simulink model "Sensores_Reales_2"  (R2026b)
settings: Solver=VariableStepAuto
values from neighbouring files (symbols this model uses):
  tau_RTD = %g s.\n',      base.wn_E,base.wn_I,base.wn_V,base.tau_RTD)    [barrido_filtros_reales.m]    (also in coeficientes.m = 20)
  wn_E = 6000    [coeficientes.m]
  wn_I = 2*6000    (= 12000)    [coeficientes.m]
  zeta_E = 1    [coeficientes.m]
  zeta_I = 1    [coeficientes.m]
settings Model: Creator=fedeb  LastModifiedBy=fedeb

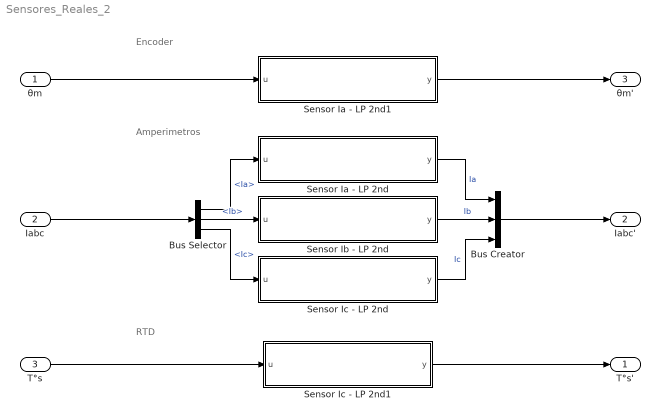
== system Sensores_Reales_2 ==
  note: RTD
  note: Amperimetros
  note: Encoder
  θm : Inport
  Iabc : Inport  Port=2
  T°s : Inport  Port=3
  Bus Creator : BusCreator  Inputs=3
  Bus Selector : BusSelector  OutputSignals=Ia,Ib,Ic
  Sensor Ia - LP 2nd : Subsystem
  Sensor Ia - LP 2nd1 : Subsystem
  Sensor Ib - LP 2nd : Subsystem
  Sensor Ic - LP 2nd : Subsystem
  Sensor Ic - LP 2nd1 : Subsystem
  T°s' : Outport
  Iabc' : Outport  Port=2
  θm' : Outport  Port=3
  wires:
  T°s/1 -> Sensor Ic - LP 2nd1/1(u)
  Sensor Ic - LP 2nd1/1(y) -> T°s'/1
  Bus Creator/1 -> Iabc'/1
  Sensor Ib - LP 2nd/1(y) -> Bus Creator/2  "Ib"
  Sensor Ia - LP 2nd/1(y) -> Bus Creator/1  "Ia"
  Bus Selector/3 -> Sensor Ic - LP 2nd/1(u)  "<Ic>"
  Bus Selector/2 -> Sensor Ib - LP 2nd/1(u)  "<Ib>"
  Sensor Ia - LP 2nd1/1(y) -> θm'/1
  Sensor Ic - LP 2nd/1(y) -> Bus Creator/3  "Ic"
  Bus Selector/1 -> Sensor Ia - LP 2nd/1(u)  "<Ia>"
  θm/1 -> Sensor Ia - LP 2nd1/1(u)
  Iabc/1 -> Bus Selector/1

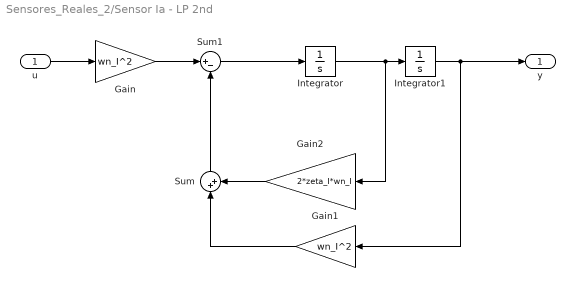
== system Sensores_Reales_2/Sensor Ia - LP 2nd ==
  u : Inport
  Gain : Gain  Gain=wn_I^2
  Gain1 : Gain  Gain=wn_I^2
  Gain2 : Gain  Gain=2*zeta_I*wn_I
  Integrator : Integrator
  Integrator1 : Integrator
  Sum : Sum  Inputs=|++
  Sum1 : Sum  Inputs=|+-
  y : Outport
  wires:
  u/1 -> Gain/1
  Gain/1 -> Sum1/1
  Sum/1 -> Sum1/2
  Sum1/1 -> Integrator/1
  Gain2/1 -> Sum/2
  Gain1/1 -> Sum/1
  Integrator/1 -> Gain2/1, Integrator1/1
  Integrator1/1 -> Gain1/1, y/1

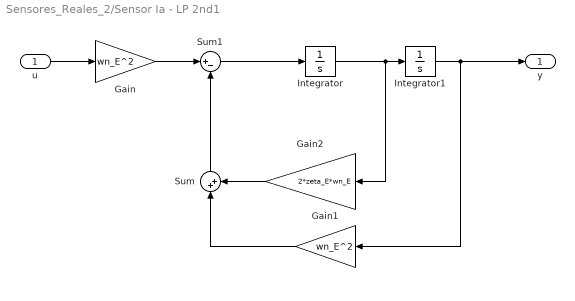
== system Sensores_Reales_2/Sensor Ia - LP 2nd1 ==
  u : Inport
  Gain : Gain  Gain=wn_E^2
  Gain1 : Gain  Gain=wn_E^2
  Gain2 : Gain  Gain=2*zeta_E*wn_E
  Integrator : Integrator
  Integrator1 : Integrator
  Sum : Sum  Inputs=|++
  Sum1 : Sum  Inputs=|+-
  y : Outport
  wires:
  Integrator1/1 -> y/1, Gain1/1
  Integrator/1 -> Integrator1/1, Gain2/1
  Gain1/1 -> Sum/1
  Gain2/1 -> Sum/2
  Sum1/1 -> Integrator/1
  Sum/1 -> Sum1/2
  Gain/1 -> Sum1/1
  u/1 -> Gain/1

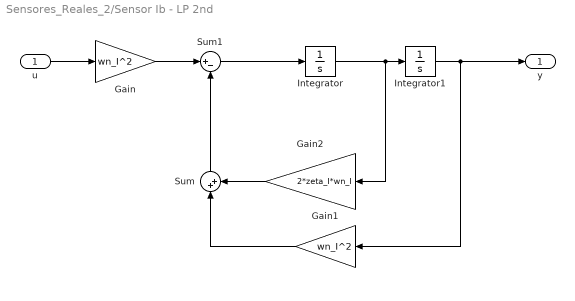
== system Sensores_Reales_2/Sensor Ib - LP 2nd ==
  u : Inport
  Gain : Gain  Gain=wn_I^2
  Gain1 : Gain  Gain=wn_I^2
  Gain2 : Gain  Gain=2*zeta_I*wn_I
  Integrator : Integrator
  Integrator1 : Integrator
  Sum : Sum  Inputs=|++
  Sum1 : Sum  Inputs=|+-
  y : Outport
  wires:
  Integrator1/1 -> y/1, Gain1/1
  Integrator/1 -> Integrator1/1, Gain2/1
  Gain1/1 -> Sum/1
  Gain2/1 -> Sum/2
  Sum1/1 -> Integrator/1
  Sum/1 -> Sum1/2
  Gain/1 -> Sum1/1
  u/1 -> Gain/1

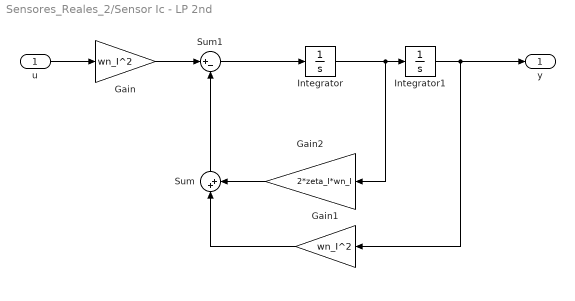
== system Sensores_Reales_2/Sensor Ic - LP 2nd ==
  u : Inport
  Gain : Gain  Gain=wn_I^2
  Gain1 : Gain  Gain=wn_I^2
  Gain2 : Gain  Gain=2*zeta_I*wn_I
  Integrator : Integrator
  Integrator1 : Integrator
  Sum : Sum  Inputs=|++
  Sum1 : Sum  Inputs=|+-
  y : Outport
  wires:
  u/1 -> Gain/1
  Gain/1 -> Sum1/1
  Sum/1 -> Sum1/2
  Sum1/1 -> Integrator/1
  Gain2/1 -> Sum/2
  Gain1/1 -> Sum/1
  Integrator/1 -> Gain2/1, Integrator1/1
  Integrator1/1 -> Gain1/1, y/1

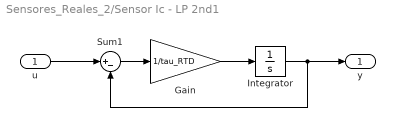
== system Sensores_Reales_2/Sensor Ic - LP 2nd1 ==
  u : Inport
  Gain : Gain  Gain=1/tau_RTD
  Integrator : Integrator
  Sum1 : Sum  Inputs=|+-
  y : Outport
  wires:
  Sum1/1 -> Gain/1
  u/1 -> Sum1/1
  Integrator/1 -> Sum1/2, y/1
  Gain/1 -> Integrator/1
